simulink model "Inverter2_senaryo1_R2025b_baseline_selected_common_dsei_precharged_raw_5ms"  (R2025b)
settings: Solver=ode23t  StartTime=0.0  StopTime=0.005  MaxStep=1e-7  EnableMultiTasking=on
PreLoadFcn:
  | irradiance = 1000;
  | i_ac_ref = 20.05;
  | v_dc_ref = 342;
  | temperature = 20;
  | f_pwm = 10000;
  | L = 0.005;
  | C = 5000e-6;
  | ts = 1/f_pwm/10;
  | v_ac_nom = 110;
libraries: ee_lib x39, fl_lib x31, nesl_utility x16, eeGeneralControl x3, eePowerMeasurement x1, eeRmsMeasurement x1, eeTotalHarmonicDistorsion x1
(part 2 of 2)

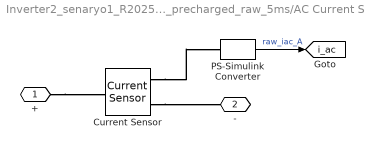
== system Inverter2_senaryo1_R2025b_baseline_selected_common_dsei_precharged_raw_5ms/AC Current Sensor1 ==
  Current Sensor : fl_lib/Electrical/Electrical Sensors/Current Sensor
  PS-Simulink Converter : nesl_utility/PS-Simulink Converter  PhysicalDomain=network_engine_domain  SubClassName=ps_output  LeftPortType=input  RightPortType=output  PseudoPeriodic=off  Frequencies=[]  VectorFormat=1-D array  Unit=1  AffineConversion=off
  + : PMIOPort  Side=Right
  - : PMIOPort  Port=2  Side=Right
  tag scope: i_ac=global
  wires:
  PS-Simulink Converter/1 -> [i_ac]  "raw_iac_A"
  connections:
  Current Sensor/RConn1 -- PS-Simulink Converter/LConn1
  +/RConn1 -- Current Sensor/LConn1
  Current Sensor/RConn2 -- -/RConn1

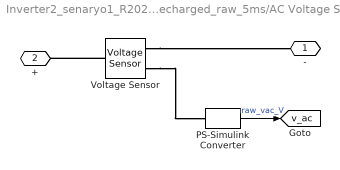
== system Inverter2_senaryo1_R2025b_baseline_selected_common_dsei_precharged_raw_5ms/AC Voltage Sensor1 ==
  PS-Simulink Converter : nesl_utility/PS-Simulink Converter  PhysicalDomain=network_engine_domain  SubClassName=ps_output  LeftPortType=input  RightPortType=output  PseudoPeriodic=off  Frequencies=[]  VectorFormat=1-D array  Unit=1  AffineConversion=off
  Voltage Sensor : fl_lib/Electrical/Electrical Sensors/Voltage Sensor
  - : PMIOPort  Side=Left
  + : PMIOPort  Port=2  Side=Right
  tag scope: v_ac=global
  wires:
  PS-Simulink Converter/1 -> [v_ac]  "raw_vac_V"
  connections:
  Voltage Sensor/RConn2 -- -/RConn1
  Voltage Sensor/RConn1 -- PS-Simulink Converter/LConn1
  Voltage Sensor/LConn1 -- +/RConn1

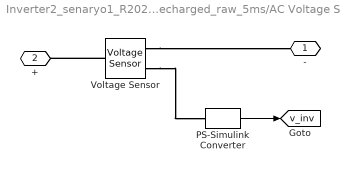
== system Inverter2_senaryo1_R2025b_baseline_selected_common_dsei_precharged_raw_5ms/AC Voltage Sensor2 ==
  PS-Simulink Converter : nesl_utility/PS-Simulink Converter  PhysicalDomain=network_engine_domain  SubClassName=ps_output  LeftPortType=input  RightPortType=output  PseudoPeriodic=off  Frequencies=[]  VectorFormat=1-D array  Unit=1  AffineConversion=off
  Voltage Sensor : fl_lib/Electrical/Electrical Sensors/Voltage Sensor
  - : PMIOPort  Side=Left
  + : PMIOPort  Port=2  Side=Right
  tag scope: v_inv=global
  wires:
  PS-Simulink Converter/1 -> [v_inv]
  connections:
  Voltage Sensor/LConn1 -- +/RConn1
  Voltage Sensor/RConn1 -- PS-Simulink Converter/LConn1
  Voltage Sensor/RConn2 -- -/RConn1

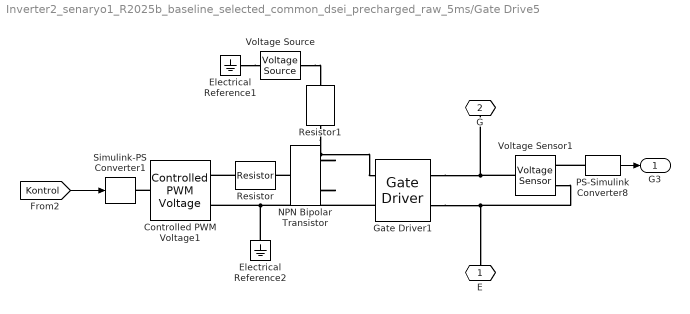
== system Inverter2_senaryo1_R2025b_baseline_selected_common_dsei_precharged_raw_5ms/Gate Drive5 ==
  Controlled PWM Voltage1 : ee_lib/Integrated Circuits/Controlled PWM Voltage  F=10 kHz  TD=0 us  pulse_width_offset=0 us  pulse_min=0 s  pwm_or_av=1  event_type=1  sample_time=1/f_pwm/100 s  Vmin=0 V  Vmax=5 V  Vm=5 V  u_min=0  u_max=1
      settings: InternalSimscapePortConfiguration="{\"Bottom\":[],\"Left\":[{\"id\":\"u\",\"label\":\"u\",\"type\":\"input\"}],\"Right\":[{\"id\":\"p2\",\"label\":\"PWM\",\"type\":\"foundation.electrical.electrical\"},{\"id\":\"n2\",\"label\":\"REF\",\"type\":\"foundation.electrical.electrical\"}],\"Top\":[]}"
  Electrical Reference1 : fl_lib/Electrical/Electrical Elements/Electrical Reference
  Electrical Reference2 : fl_lib/Electrical/Electrical Elements/Electrical Reference
  Gate Driver1 : ee_lib/Semiconductors & Converters/Gate Driver  port_option=ee.enum.controlport.elec  uHigh=4 V  uLow=3 V  uHighValue=0.7  uLowValue=0.3  vHigh=15 V  vLow=-5 V  tHigh=4 us  tLow=0 us  parameterization=1  rHigh=10 Ohm  rLow=10 Ohm  tRise=20 ns  tFall=20 ns  cLoad=10 nF  ZonTime_specify=off  ZonTime_priority=None  ZonTime=0 s  ZoffTime_specify=off  ZoffTime_priority=None  ZoffTime=0 s
  NPN Bipolar Transistor : ee_lib/Semiconductors & Converters/NPN Bipolar Transistor  parameterization=1  BF=100  IS=1e-14 A  VAF=200 V  hfe=100  hoe=50e-6 1/Ohm  Ic_h=1 mA  Vce_h=5 V  V1=0.55 V  I1=0.5 mA  BR=1  Tmeas=25 degC  RC=0.01 Ohm  RE=1e-4 Ohm  RB=1 Ohm  C_BC=5 pF  C_BE=5 pF  TF=0 us  TR=0 us  prmDatasheet=1  prmEquCoeff=1  hfe_T2=125  XTB=0  V1_T2=0.45 V  I1_T2=0.5 mA  Tmeas2=125 degC  EG=1.11 eV  XTI=3  TdeviceDatasheet=25 degC  TdeviceEquCoeff=25 degC  ec=1  ib_specify=off  ib_priority=None  ib=0 A  ib_nominal_specify=off  ib_nominal_value=1  ib_nominal_unit=A  ic_specify=off  ic_priority=None  ic=0 A  ic_nominal_specify=off  ic_nominal_value=1  ic_nominal_unit=A  vce_specify=off  vce_priority=None  vce=0 V  vce_nominal_specify=off  vce_nominal_value=1  vce_nominal_unit=V  vbe_specify=off  vbe_priority=None  vbe=0 V  vbe_nominal_specify=off  vbe_nominal_value=1  vbe_nominal_unit=V  Qbc_specify=off  Qbc_priority=High  Qbc=0 C  Qbc_nominal_specify=off  Qbc_nominal_value=1  Qbc_nominal_unit=uC  Qbe_specify=off  Qbe_priority=High  Qbe=0 C  Qbe_nominal_specify=off  Qbe_nominal_value=1  Qbe_nominal_unit=uC  thermal_network_parameterization=ee.enum.thermalNetworkTopology.junctionCase  Rth=[0, 10] K/W  Rth_Cauer=[1, 3, 10] K/W  Rth_Foster=[4, 6] K/W  thermal_mass_parameterization=ee.enum.thermalNetwork.timeconstant  thermal_mass=[0, 1] J/K  thermal_mass_Cauer=[.1, .3, 1] J/K  thermal_mass_Foster=[1.5, 3] J/K  thermal_time_constant=[0, 10] s  thermal_time_constant_Cauer=[1, 3, 10] s  thermal_time_constant_Foster=[6, 18] s  thermal_mass_initial_temperatures=[25, 25] degC  thermal_mass_initial_temperatures_Cauer=[25, 25, 25] degC  Tvec_initial_Foster=[25, 25, 25, 25] degC
      settings: InternalSimscapePortConfiguration="{\"Bottom\":[],\"Left\":[{\"id\":\"B\",\"label\":\"\",\"type\":\"foundation.electrical.electrical\"}],\"Right\":[{\"id\":\"C\",\"label\":\"\",\"type\":\"foundation.electrical.electrical\"},{\"id\":\"E\",\"label\":\"\",\"type\":\"foundation.electrical.electrical\"}],\"Top\":[]}"
  PS-Simulink Converter8 : nesl_utility/PS-Simulink Converter  PhysicalDomain=network_engine_domain  SubClassName=ps_output  LeftPortType=input  RightPortType=output  PseudoPeriodic=off  Frequencies=[]  VectorFormat=1-D array  Unit=1  AffineConversion=off
  Resistor : ee_lib/Passive/Resistor  R=1 kOhm  enable_R_tol=ee.enum.toleranceApplication.none  R_tol=5  tol_distribution=ee.enum.toleranceDistribution.uniform  nSigma=4  enable_operating_limits=ee.enum.enable.no  operating_limit_action=ee.enum.passive.reportOpLim.warn  power_rating=1 W  max_working_voltage=100 V  noise_mode=ee.enum.sources.noise.Disabled  Tdevice=25 degC  sample_time=1e-3 s  repeatability=ee.enum.ic.repeatability.notRepeatable  user_seed=0  auto_seed=4111000739  power_derating_T1=70 degC  power_derating_T2=155 degC  operating_temperature_range_vec=[-50, 150] degC  alpha=3.93e-3 1/K  Tmeas=25 degC  thermal_mass=100 J/K  temperature_specify=off  temperature_priority=High  temperature=298.15 K  temperature_nominal_specify=off  temperature_nominal_value=1  temperature_nominal_unit=K
  Resistor1 : ee_lib/Passive/Resistor  R=1 kOhm  enable_R_tol=ee.enum.toleranceApplication.none  R_tol=5  tol_distribution=ee.enum.toleranceDistribution.uniform  nSigma=4  enable_operating_limits=ee.enum.enable.no  operating_limit_action=ee.enum.passive.reportOpLim.warn  power_rating=1 W  max_working_voltage=100 V  noise_mode=ee.enum.sources.noise.Disabled  Tdevice=25 degC  sample_time=1e-3 s  repeatability=ee.enum.ic.repeatability.notRepeatable  user_seed=0  auto_seed=2084672538  power_derating_T1=70 degC  power_derating_T2=155 degC  operating_temperature_range_vec=[-50, 150] degC  alpha=3.93e-3 1/K  Tmeas=25 degC  thermal_mass=100 J/K  temperature_specify=off  temperature_priority=High  temperature=298.15 K  temperature_nominal_specify=off  temperature_nominal_value=1  temperature_nominal_unit=K
  Simulink-PS Converter1 : nesl_utility/Simulink-PS Converter  PhysicalDomain=network_engine_domain  SubClassName=ps_input  LeftPortType=input  RightPortType=output  PseudoPeriodic=off  Frequencies=[]  NoiseDistribution=none  NoiseParameters=[]  Unit=1  AffineConversion=off  FilteringAndDerivatives=zero  SimscapeFilterOrder=1  InputFilterTimeConstant=0.001  UdotUserProvided=1
  Voltage Sensor1 : fl_lib/Electrical/Electrical Sensors/Voltage Sensor
  Voltage Source : ee_lib/Sources/Voltage Source  dc_voltage=5 V  ac_voltage=0 V  ac_shift=0 rad  ac_frequency=60 Hz  noise_mode=ee.enum.sources.noise.Disabled  PSD=0 V^2/Hz  sample_time=1e-3 s  repeatability=ee.enum.sources.repeatability.NotRepeatable  user_seed=0  auto_seed=3437178441  i_specify=off  i_priority=None  i=0 A  i_nominal_specify=off  i_nominal_value=1  i_nominal_unit=A  v_specify=off  v_priority=None  v=0 V  v_nominal_specify=off  v_nominal_value=1  v_nominal_unit=V
  E : PMIOPort  Side=Right
  G : PMIOPort  Port=2  Side=Right
  G3 : Outport  VectorParamsAs1DForOutWhenUnconnected=off
  wires:
  [Kontrol] -> Simulink-PS Converter1/1
  PS-Simulink Converter8/1 -> G3/1
  connections:
  Gate Driver1/RConn2 -- Voltage Sensor1/RConn2 -- E/RConn1
  Gate Driver1/RConn1 -- Voltage Sensor1/LConn1 -- G/RConn1
  Controlled PWM Voltage1/LConn1 -- Simulink-PS Converter1/RConn1
  Electrical Reference2/LConn1 -- Gate Driver1/LConn2 -- NPN Bipolar Transistor/RConn2 -- Controlled PWM Voltage1/RConn2
  NPN Bipolar Transistor/LConn1 -- Resistor/RConn1
  Resistor/LConn1 -- Controlled PWM Voltage1/RConn1
  NPN Bipolar Transistor/RConn1 -- Resistor1/RConn1 -- Gate Driver1/LConn1
  Voltage Source/LConn1 -- Resistor1/LConn1
  PS-Simulink Converter8/LConn1 -- Voltage Sensor1/RConn1
  Electrical Reference1/LConn1 -- Voltage Source/RConn1

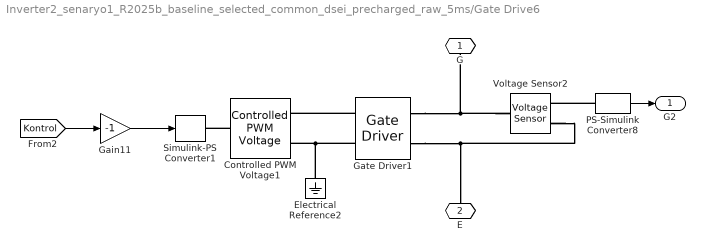
== system Inverter2_senaryo1_R2025b_baseline_selected_common_dsei_precharged_raw_5ms/Gate Drive6 ==
  Controlled PWM Voltage1 : ee_lib/Integrated Circuits/Controlled PWM Voltage  F=10 kHz  TD=0 us  pulse_width_offset=0 s  pulse_min=0 s  pwm_or_av=1  event_type=1  sample_time=1/f_pwm/100 s  Vmin=0 V  Vmax=5 V  Vm=5 V  u_min=0  u_max=1
      settings: InternalSimscapePortConfiguration="{\"Bottom\":[],\"Left\":[{\"id\":\"u\",\"label\":\"u\",\"type\":\"input\"}],\"Right\":[{\"id\":\"p2\",\"label\":\"PWM\",\"type\":\"foundation.electrical.electrical\"},{\"id\":\"n2\",\"label\":\"REF\",\"type\":\"foundation.electrical.electrical\"}],\"Top\":[]}"
  Electrical Reference2 : fl_lib/Electrical/Electrical Elements/Electrical Reference
  Gain11 : Gain  Gain=-1
  Gate Driver1 : ee_lib/Semiconductors & Converters/Gate Driver  port_option=ee.enum.controlport.elec  uHigh=4 V  uLow=3 V  uHighValue=0.7  uLowValue=0.3  vHigh=15 V  vLow=-5 V  tHigh=4 us  tLow=0 ns  parameterization=1  rHigh=10 Ohm  rLow=10 Ohm  tRise=20 ns  tFall=20 ns  cLoad=10 nF  ZonTime_specify=off  ZonTime_priority=None  ZonTime=0 s  ZoffTime_specify=off  ZoffTime_priority=None  ZoffTime=0 s
  PS-Simulink Converter8 : nesl_utility/PS-Simulink Converter  PhysicalDomain=network_engine_domain  SubClassName=ps_output  LeftPortType=input  RightPortType=output  PseudoPeriodic=off  Frequencies=[]  VectorFormat=1-D array  Unit=1  AffineConversion=off
  Simulink-PS Converter1 : nesl_utility/Simulink-PS Converter  PhysicalDomain=network_engine_domain  SubClassName=ps_input  LeftPortType=input  RightPortType=output  PseudoPeriodic=off  Frequencies=[]  NoiseDistribution=none  NoiseParameters=[]  Unit=1  AffineConversion=off  FilteringAndDerivatives=zero  SimscapeFilterOrder=1  InputFilterTimeConstant=0.001  UdotUserProvided=1
  Voltage Sensor2 : fl_lib/Electrical/Electrical Sensors/Voltage Sensor
  G : PMIOPort  Side=Right
  E : PMIOPort  Port=2  Side=Right
  G2 : Outport  VectorParamsAs1DForOutWhenUnconnected=off
  wires:
  Gain11/1 -> Simulink-PS Converter1/1
  [Kontrol] -> Gain11/1
  PS-Simulink Converter8/1 -> G2/1
  connections:
  Gate Driver1/RConn2 -- Voltage Sensor2/RConn2 -- E/RConn1
  Gate Driver1/RConn1 -- Voltage Sensor2/LConn1 -- G/RConn1
  Controlled PWM Voltage1/LConn1 -- Simulink-PS Converter1/RConn1
  Gate Driver1/LConn1 -- Controlled PWM Voltage1/RConn1
  Electrical Reference2/LConn1 -- Controlled PWM Voltage1/RConn2 -- Gate Driver1/LConn2
  PS-Simulink Converter8/LConn1 -- Voltage Sensor2/RConn1

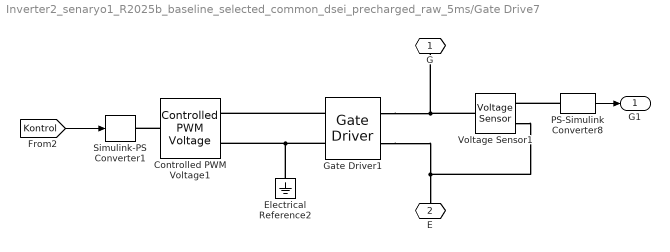
== system Inverter2_senaryo1_R2025b_baseline_selected_common_dsei_precharged_raw_5ms/Gate Drive7 ==
  Controlled PWM Voltage1 : ee_lib/Integrated Circuits/Controlled PWM Voltage  F=10 kHz  TD=0 us  pulse_width_offset=0 s  pulse_min=0 s  pwm_or_av=1  event_type=1  sample_time=1/f_pwm/100 s  Vmin=0 V  Vmax=5 V  Vm=5 V  u_min=0  u_max=1
      settings: InternalSimscapePortConfiguration="{\"Bottom\":[],\"Left\":[{\"id\":\"u\",\"label\":\"u\",\"type\":\"input\"}],\"Right\":[{\"id\":\"p2\",\"label\":\"PWM\",\"type\":\"foundation.electrical.electrical\"},{\"id\":\"n2\",\"label\":\"REF\",\"type\":\"foundation.electrical.electrical\"}],\"Top\":[]}"
  Electrical Reference2 : fl_lib/Electrical/Electrical Elements/Electrical Reference
  Gate Driver1 : ee_lib/Semiconductors & Converters/Gate Driver  port_option=ee.enum.controlport.elec  uHigh=4 V  uLow=3 V  uHighValue=0.7  uLowValue=0.3  vHigh=15 V  vLow=-5 V  tHigh=4 us  tLow=0 ns  parameterization=1  rHigh=10 Ohm  rLow=10 Ohm  tRise=20 ns  tFall=20 ns  cLoad=10 nF  ZonTime_specify=off  ZonTime_priority=None  ZonTime=0 s  ZoffTime_specify=off  ZoffTime_priority=None  ZoffTime=0 s
  PS-Simulink Converter8 : nesl_utility/PS-Simulink Converter  PhysicalDomain=network_engine_domain  SubClassName=ps_output  LeftPortType=input  RightPortType=output  PseudoPeriodic=off  Frequencies=[]  VectorFormat=1-D array  Unit=1  AffineConversion=off
  Simulink-PS Converter1 : nesl_utility/Simulink-PS Converter  PhysicalDomain=network_engine_domain  SubClassName=ps_input  LeftPortType=input  RightPortType=output  PseudoPeriodic=off  Frequencies=[]  NoiseDistribution=none  NoiseParameters=[]  Unit=1  AffineConversion=off  FilteringAndDerivatives=zero  SimscapeFilterOrder=1  InputFilterTimeConstant=0.001  UdotUserProvided=1
  Voltage Sensor1 : fl_lib/Electrical/Electrical Sensors/Voltage Sensor
  G : PMIOPort  Side=Right
  E : PMIOPort  Port=2  Side=Right
  G1 : Outport  VectorParamsAs1DForOutWhenUnconnected=off
  wires:
  [Kontrol] -> Simulink-PS Converter1/1
  PS-Simulink Converter8/1 -> G1/1
  connections:
  Gate Driver1/LConn2 -- Electrical Reference2/LConn1 -- Controlled PWM Voltage1/RConn2
  Gate Driver1/LConn1 -- Controlled PWM Voltage1/RConn1
  Controlled PWM Voltage1/LConn1 -- Simulink-PS Converter1/RConn1
  Gate Driver1/RConn1 -- G/RConn1 -- Voltage Sensor1/LConn1
  Gate Driver1/RConn2 -- Voltage Sensor1/RConn2 -- E/RConn1
  PS-Simulink Converter8/LConn1 -- Voltage Sensor1/RConn1

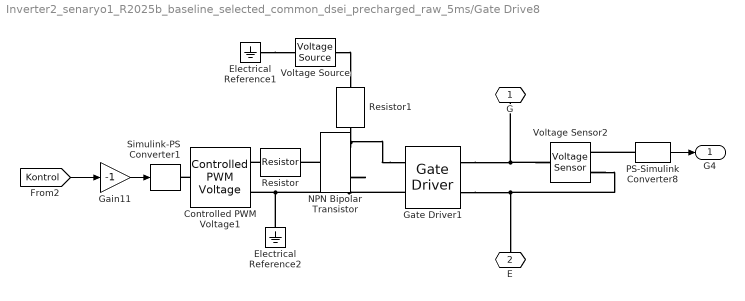
== system Inverter2_senaryo1_R2025b_baseline_selected_common_dsei_precharged_raw_5ms/Gate Drive8 ==
  Controlled PWM Voltage1 : ee_lib/Integrated Circuits/Controlled PWM Voltage  F=10 kHz  TD=0 us  pulse_width_offset=0 us  pulse_min=0 s  pwm_or_av=1  event_type=1  sample_time=1/f_pwm/100 s  Vmin=0 V  Vmax=5 V  Vm=5 V  u_min=0  u_max=1
      settings: InternalSimscapePortConfiguration="{\"Bottom\":[],\"Left\":[{\"id\":\"u\",\"label\":\"u\",\"type\":\"input\"}],\"Right\":[{\"id\":\"p2\",\"label\":\"PWM\",\"type\":\"foundation.electrical.electrical\"},{\"id\":\"n2\",\"label\":\"REF\",\"type\":\"foundation.electrical.electrical\"}],\"Top\":[]}"
  Electrical Reference1 : fl_lib/Electrical/Electrical Elements/Electrical Reference
  Electrical Reference2 : fl_lib/Electrical/Electrical Elements/Electrical Reference
  Gain11 : Gain  Gain=-1
  Gate Driver1 : ee_lib/Semiconductors & Converters/Gate Driver  port_option=ee.enum.controlport.elec  uHigh=4 V  uLow=3 V  uHighValue=0.7  uLowValue=0.3  vHigh=15 V  vLow=-5 V  tHigh=4 us  tLow=0 us  parameterization=1  rHigh=10 Ohm  rLow=10 Ohm  tRise=20 ns  tFall=20 ns  cLoad=10 nF  ZonTime_specify=off  ZonTime_priority=None  ZonTime=0 s  ZoffTime_specify=off  ZoffTime_priority=None  ZoffTime=0 s
  NPN Bipolar Transistor : ee_lib/Semiconductors & Converters/NPN Bipolar Transistor  parameterization=1  BF=100  IS=1e-14 A  VAF=200 V  hfe=100  hoe=50e-6 1/Ohm  Ic_h=1 mA  Vce_h=5 V  V1=0.55 V  I1=0.5 mA  BR=1  Tmeas=25 degC  RC=0.01 Ohm  RE=1e-4 Ohm  RB=1 Ohm  C_BC=5 pF  C_BE=5 pF  TF=0 us  TR=0 us  prmDatasheet=1  prmEquCoeff=1  hfe_T2=125  XTB=0  V1_T2=0.45 V  I1_T2=0.5 mA  Tmeas2=125 degC  EG=1.11 eV  XTI=3  TdeviceDatasheet=25 degC  TdeviceEquCoeff=25 degC  ec=1  ib_specify=off  ib_priority=None  ib=0 A  ib_nominal_specify=off  ib_nominal_value=1  ib_nominal_unit=A  ic_specify=off  ic_priority=None  ic=0 A  ic_nominal_specify=off  ic_nominal_value=1  ic_nominal_unit=A  vce_specify=off  vce_priority=None  vce=0 V  vce_nominal_specify=off  vce_nominal_value=1  vce_nominal_unit=V  vbe_specify=off  vbe_priority=None  vbe=0 V  vbe_nominal_specify=off  vbe_nominal_value=1  vbe_nominal_unit=V  Qbc_specify=off  Qbc_priority=High  Qbc=0 C  Qbc_nominal_specify=off  Qbc_nominal_value=1  Qbc_nominal_unit=uC  Qbe_specify=off  Qbe_priority=High  Qbe=0 C  Qbe_nominal_specify=off  Qbe_nominal_value=1  Qbe_nominal_unit=uC  thermal_network_parameterization=ee.enum.thermalNetworkTopology.junctionCase  Rth=[0, 10] K/W  Rth_Cauer=[1, 3, 10] K/W  Rth_Foster=[4, 6] K/W  thermal_mass_parameterization=ee.enum.thermalNetwork.timeconstant  thermal_mass=[0, 1] J/K  thermal_mass_Cauer=[.1, .3, 1] J/K  thermal_mass_Foster=[1.5, 3] J/K  thermal_time_constant=[0, 10] s  thermal_time_constant_Cauer=[1, 3, 10] s  thermal_time_constant_Foster=[6, 18] s  thermal_mass_initial_temperatures=[25, 25] degC  thermal_mass_initial_temperatures_Cauer=[25, 25, 25] degC  Tvec_initial_Foster=[25, 25, 25, 25] degC
      settings: InternalSimscapePortConfiguration="{\"Bottom\":[],\"Left\":[{\"id\":\"B\",\"label\":\"\",\"type\":\"foundation.electrical.electrical\"}],\"Right\":[{\"id\":\"C\",\"label\":\"\",\"type\":\"foundation.electrical.electrical\"},{\"id\":\"E\",\"label\":\"\",\"type\":\"foundation.electrical.electrical\"}],\"Top\":[]}"
  PS-Simulink Converter8 : nesl_utility/PS-Simulink Converter  PhysicalDomain=network_engine_domain  SubClassName=ps_output  LeftPortType=input  RightPortType=output  PseudoPeriodic=off  Frequencies=[]  VectorFormat=1-D array  Unit=1  AffineConversion=off
  Resistor : ee_lib/Passive/Resistor  R=1 kOhm  enable_R_tol=ee.enum.toleranceApplication.none  R_tol=5  tol_distribution=ee.enum.toleranceDistribution.uniform  nSigma=4  enable_operating_limits=ee.enum.enable.no  operating_limit_action=ee.enum.passive.reportOpLim.warn  power_rating=1 W  max_working_voltage=100 V  noise_mode=ee.enum.sources.noise.Disabled  Tdevice=25 degC  sample_time=1e-3 s  repeatability=ee.enum.ic.repeatability.notRepeatable  user_seed=0  auto_seed=3922919431  power_derating_T1=70 degC  power_derating_T2=155 degC  operating_temperature_range_vec=[-50, 150] degC  alpha=3.93e-3 1/K  Tmeas=25 degC  thermal_mass=100 J/K  temperature_specify=off  temperature_priority=High  temperature=298.15 K  temperature_nominal_specify=off  temperature_nominal_value=1  temperature_nominal_unit=K
  Resistor1 : ee_lib/Passive/Resistor  R=1 kOhm  enable_R_tol=ee.enum.toleranceApplication.none  R_tol=5  tol_distribution=ee.enum.toleranceDistribution.uniform  nSigma=4  enable_operating_limits=ee.enum.enable.no  operating_limit_action=ee.enum.passive.reportOpLim.warn  power_rating=1 W  max_working_voltage=100 V  noise_mode=ee.enum.sources.noise.Disabled  Tdevice=25 degC  sample_time=1e-3 s  repeatability=ee.enum.ic.repeatability.notRepeatable  user_seed=0  auto_seed=2715962282  power_derating_T1=70 degC  power_derating_T2=155 degC  operating_temperature_range_vec=[-50, 150] degC  alpha=3.93e-3 1/K  Tmeas=25 degC  thermal_mass=100 J/K  temperature_specify=off  temperature_priority=High  temperature=298.15 K  temperature_nominal_specify=off  temperature_nominal_value=1  temperature_nominal_unit=K
  Simulink-PS Converter1 : nesl_utility/Simulink-PS Converter  PhysicalDomain=network_engine_domain  SubClassName=ps_input  LeftPortType=input  RightPortType=output  PseudoPeriodic=off  Frequencies=[]  NoiseDistribution=none  NoiseParameters=[]  Unit=1  AffineConversion=off  FilteringAndDerivatives=zero  SimscapeFilterOrder=1  InputFilterTimeConstant=0.001  UdotUserProvided=1
  Voltage Sensor2 : fl_lib/Electrical/Electrical Sensors/Voltage Sensor
  Voltage Source : ee_lib/Sources/Voltage Source  dc_voltage=5 V  ac_voltage=0 V  ac_shift=0 rad  ac_frequency=60 Hz  noise_mode=ee.enum.sources.noise.Disabled  PSD=0 V^2/Hz  sample_time=1e-3 s  repeatability=ee.enum.sources.repeatability.NotRepeatable  user_seed=0  auto_seed=418932850  i_specify=off  i_priority=None  i=0 A  i_nominal_specify=off  i_nominal_value=1  i_nominal_unit=A  v_specify=off  v_priority=None  v=0 V  v_nominal_specify=off  v_nominal_value=1  v_nominal_unit=V
  G : PMIOPort  Side=Right
  E : PMIOPort  Port=2  Side=Right
  G4 : Outport  VectorParamsAs1DForOutWhenUnconnected=off
  wires:
  [Kontrol] -> Gain11/1
  Gain11/1 -> Simulink-PS Converter1/1
  PS-Simulink Converter8/1 -> G4/1
  connections:
  Gate Driver1/LConn1 -- NPN Bipolar Transistor/RConn1 -- Resistor1/RConn1
  Gate Driver1/LConn2 -- NPN Bipolar Transistor/RConn2 -- Electrical Reference2/LConn1 -- Controlled PWM Voltage1/RConn2
  Gate Driver1/RConn1 -- Voltage Sensor2/LConn1 -- G/RConn1
  Gate Driver1/RConn2 -- E/RConn1 -- Voltage Sensor2/RConn2
  Resistor/LConn1 -- Controlled PWM Voltage1/RConn1
  Voltage Source/LConn1 -- Resistor1/LConn1
  NPN Bipolar Transistor/LConn1 -- Resistor/RConn1
  Controlled PWM Voltage1/LConn1 -- Simulink-PS Converter1/RConn1
  PS-Simulink Converter8/LConn1 -- Voltage Sensor2/RConn1
  Electrical Reference1/LConn1 -- Voltage Source/RConn1

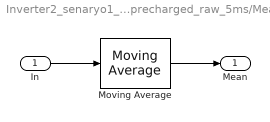
== system Inverter2_senaryo1_R2025b_baseline_selected_common_dsei_precharged_raw_5ms/Mean1 ==
  In : Inport
  Moving Average : eeGeneralControl/Moving Average  VariantControl=Variant1  LabelModeActiveChoice=Continuous  f=50  x0=0.0001  BufferSize=8192  Ts=0
  Mean : Outport  VectorParamsAs1DForOutWhenUnconnected=off
  wires:
  Moving Average/1 -> Mean/1
  In/1 -> Moving Average/1

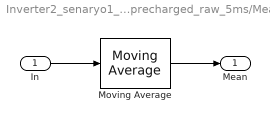
== system Inverter2_senaryo1_R2025b_baseline_selected_common_dsei_precharged_raw_5ms/Mean2 ==
  In : Inport
  Moving Average : eeGeneralControl/Moving Average  VariantControl=Variant1  LabelModeActiveChoice=Continuous  f=50  x0=0.0001  BufferSize=8192  Ts=0
  Mean : Outport  VectorParamsAs1DForOutWhenUnconnected=off
  wires:
  Moving Average/1 -> Mean/1
  In/1 -> Moving Average/1

== system Inverter2_senaryo1_R2025b_baseline_selected_common_dsei_precharged_raw_5ms/Mean3 ==
  In : Inport
  Moving Average : eeGeneralControl/Moving Average  VariantControl=Variant1  LabelModeActiveChoice=Continuous  f=50  x0=0.0001  BufferSize=8192  Ts=0
  Mean : Outport  VectorParamsAs1DForOutWhenUnconnected=off
  wires:
  Moving Average/1 -> Mean/1
  In/1 -> Moving Average/1

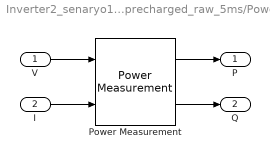
== system Inverter2_senaryo1_R2025b_baseline_selected_common_dsei_precharged_raw_5ms/Power1 ==
  V : Inport
  I : Inport  Port=2
  Power Measurement : eePowerMeasurement/Power Measurement  LabelModeActiveChoice=Continuous  F=50  K=1  Ts=0
  P : Outport  VectorParamsAs1DForOutWhenUnconnected=off
  Q : Outport  Port=2  VectorParamsAs1DForOutWhenUnconnected=off
  wires:
  Power Measurement/2 -> Q/1
  I/1 -> Power Measurement/2
  Power Measurement/1 -> P/1
  V/1 -> Power Measurement/1

== system Inverter2_senaryo1_R2025b_baseline_selected_common_dsei_precharged_raw_5ms/RMS1 ==
  In : Inport
  RMS Measurement : eeRmsMeasurement/RMS Measurement  LabelModeActiveChoice=Total  F=60  SpecifyHarmonics=off  K=[0 1 2]  Ts=0
  RMS : Outport  VectorParamsAs1DForOutWhenUnconnected=off
  wires:
  RMS Measurement/1 -> RMS/1
  In/1 -> RMS Measurement/1

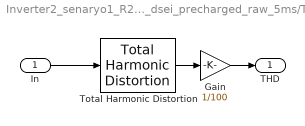
== system Inverter2_senaryo1_R2025b_baseline_selected_common_dsei_precharged_raw_5ms/THD ==
  In : Inport
  Gain : Gain  Gain=1/100  SampleTime=0
  Total Harmonic Distortion : eeTotalHarmonicDistorsion/Total Harmonic Distortion  f=50  Ts=0
  THD : Outport  VectorParamsAs1DForOutWhenUnconnected=off
  wires:
  Gain/1 -> THD/1
  In/1 -> Total Harmonic Distortion/1
  Total Harmonic Distortion/1 -> Gain/1
